simulink model "jumeau_banc_rw"  (R2025b)
settings: Solver=ode23t  StartTime=0.0  StopTime=20  MaxStep=1e-3  RelTol=1e-4
PostLoadFcn:
  | d = fileparts(get_param('jumeau_banc_rw', 'FileName')); addpath(fullfile(d, 'geometrie'), fullfile(d, 'liaison'), fullfile(d, 'pilotage')); clear d
StartFcn:
  | % Jumeau Webots : au lancement, MATLAB envoie les paramètres du Model Workspace à Webots, qui remet le banc en
  | % position de départ, puis ouvre la liaison de télémétrie et la liaison de commande (liaison/pont_banc.m).
  | if strcmp(get_param('jumeau_banc_rw/Procédé', 'LabelModeActiveChoice'), 'Webots')
  |     pont_banc('ouvrir', getVariable(get_param('jumeau_banc_rw', 'ModelWorkspace'), 'config_jumeau'));
  | end
  | pilotage_banc('depart');   % interface de pilotage : nouveau lancement
StopFcn:
  | pont_banc('fermer');
  | pilotage_banc('fin');
model workspace (MATLAB code in the model file):
  | %% Jumeau numérique du banc de stabilisation à 4 roues de réaction (version 3) : paramètres
  | % Ce code est enregistré dans le modèle (Model Explorer > jumeau_banc_rw > Model Workspace).
  | % Origine : (CAO) CAO du banc version 3, (M) mesuré sur le matériel, (F) fiche technique, (Fw) firmware,
  | % (H) hypothèse à mesurer sur le banc. Masses et inerties des pièces : dans chaque bloc de pièce.
  | 
  | %% Montage de l'essai
  | pivot_mm = 25;              % position du pivot de tangage sur le corps : 25, 24, 16, 8, 0, -8 mm (25 : banc équilibré, rangée +24 et paliers remontés de 1 mm)
  | blocage_roulis = 0;         % goupille de blocage : 1 = axe bloqué à 0°, 0 = axe libre
  | blocage_tangage = 0;
  | angle0_roulis_deg = 2;      % position de départ (mise à 0 si l'axe est bloqué)
  | angle0_tangage_deg = -1;
  | g = 9.81;                   % m/s²
  | 
  | %% Pupitre : pilotage manuel des 4 ESC
  | essai_t = 1;                % s, instant de l'échelon d'essai ajouté aux curseurs
  | essai_echelon_us = [0 0 0 0];   % µs, échelon d'essai sur chaque ESC (0 : aucun)
  | 
  | %% Alimentation des ESC
  | V_alim = 12;                % V, alimentation de labo (H : tension réglée)
  | 
  | %% ESC Brushless 30A bidirectionnels (x4)
  | f_trame_esc = 50;           % Hz, une impulsion toutes les 20 ms (Fw : LEDC 50 Hz)
  | imp_neutre = 1500;          % µs, neutre (testé sur le banc)
  | imp_min = 1000;             % µs (Fw)
  | imp_max = 2000;             % µs (Fw)
  | zone_morte_us = 0;          % µs autour du neutre (H)
  | tau_esc = 2e-3;             % s, temps de réponse de l'ESC (H)
  | armement_actif = 1;         % 1 : l'ESC ne pilote le moteur qu'après t_armement au neutre
  | t_armement = 1;             % s (H)
  | fenetre_armement_us = 25;   % µs, écart au neutre accepté pendant l'armement (H)
  | sens_moteurs = [1 1 1 1];   % +1 : au-dessus du neutre, la roue tourne dans le sens +axe (vers l'extérieur) (H : ordre des phases)
  | 
  | %% Moteurs A2212 1400 KV (x4), modèle équivalent continu
  | KV = 1400;                  % tr/min/V (F)
  | Ke = 60/(2*pi*KV);          % V.s/rad
  | Kt = Ke;                    % N.m/A
  | R_moteur = 0.08;            % ohm (H)
  | L_moteur = 30e-6;           % H (H)
  | f_roue = 5e-6;              % N.m.s/rad, frottement visqueux des roulements du moteur (H)
  | 
  | %% Cardan
  | butee_deg = 20;             % débattement de chaque axe (CAO)
  | k_butee = 20;               % N.m/rad, contact goupille-lumière (H)
  | c_butee = 0.2;              % N.m.s/rad (H)
  | b_cardan = 1e-4;            % N.m.s/rad, frottement des roulements 625 (H)
  | k_cables = 0;               % N.m/rad, raideur des deux câbles vers la table (H)
  | 
  | %% BNO055 (mode fusion)
  | T_bno = 0.01;               % s, données de fusion à 100 Hz (F)
  | bruit_bno = 1;              % 1 : bruit de mesure, 0 : capteur parfait
  | sigma_angle_deg = 0.05;     % ° (H)
  | sigma_gyro_dps = 0.1;       % °/s (H)
  | sigma_acc = 0.02;           % m/s² (H)
  | R_montage_bno = eye(3);     % axes du capteur dans le repère du dispositif : eye(3) = remappage AXIS_MAP réglé
  |                             % (la carte est tournée de 90° dans la CAO)
  | 
  | %% Capteurs de vitesse TCRT5000 (x4) : un front à chaque rayon du disque
  | n_rayons = 4;               % rayons du disque vus par tour (CAO : disque d'origine)
  | T_tcrt = 1e-3;              % s, pas de calcul du capteur (les fronts sont datés par interpolation, comme un chronomètre en µs)
  | t_arret_tcrt = 0.2;         % s sans front : la vitesse mesurée retombe à 0 (Fw, à fixer)
  | 
  | %% Pont vers le jumeau Webots (et, plus tard, vers l'ESP32 du banc réel)
  | T_pont = 0.01;              % s, une trame de commande et une trame de télémétrie toutes les 10 ms
  | 
  | %% Essai : maintien au départ et perturbation
  | t_lacher = 2;                % s, le dispositif est tenu à la main à sa position de départ jusqu'à cet instant (0 : libre dès le départ)
  | k_main = 5;                  % N.m/rad, raideur de la main qui tient le dispositif
  | c_main = 0.3;                % N.m.s/rad, son amortissement
  | perturbation_t = 7;          % s, instant de la poussée d'essai
  | perturbation_duree = 0.2;    % s
  | perturbation_couple = [0.02 0.02];   % N.m, couple de la poussée sur [roulis tangage], programmée (0 : aucune ; l'interface de pilotage en ajoute)
  | 
  | %% Grandeurs dérivées
  | assert(any(pivot_mm == [25 24 16 8 0 -8]), 'pivot_mm : 25, 24, 16, 8, 0, -8');
  | q0_deg = [angle0_roulis_deg angle0_tangage_deg] .* ([blocage_roulis blocage_tangage] == 0);
  | config_jumeau = [pivot_mm; blocage_roulis; blocage_tangage; q0_deg(:); V_alim; f_trame_esc; imp_neutre; imp_min; imp_max; ...
  |     zone_morte_us; tau_esc; armement_actif; t_armement; fenetre_armement_us; sens_moteurs(:); Ke; Kt; R_moteur; L_moteur; ...
  |     f_roue; butee_deg; k_butee; c_butee; b_cardan; k_cables; g; T_bno; bruit_bno; sigma_angle_deg; sigma_gyro_dps; ...
  |     sigma_acc; n_rayons; t_arret_tcrt; T_tcrt; R_montage_bno(:); T_pont; t_lacher; k_main; c_main];   % 51 valeurs envoyées au jumeau Webots au lancement
  | 
  | %% Commande bas niveau : une boucle de vitesse par roue, avec observateur CFO (méthode du TP2, ramenée à la vitesse)
  | J_roue = 1.562e-4;          % kg.m², inertie d'une roue autour de son axe : disque, vis, cloche du moteur (CAO)
  | T_cbn = 1/f_trame_esc;      % s, période de calcul de la commande : celle des ESC, qui ne lisent qu'une impulsion toutes les 20 ms
  | wc_roue = [10 10 10 10];    % rad/s, rapidité du suivi de vitesse de chaque roue (pôle de l'erreur en -wc)
  | wo_roue = [5 5 5 5];        % rad/s, rapidité du CFO de chaque roue (pôles en -wo et -4 wo) ; au-delà de 10, il devient instable à 20 ms
  | imp_cmd_min = 1375;         % µs, limites des impulsions commandées : vitesse conseillée des disques, 3 900 tr/min
  | imp_cmd_max = 1625;         % µs
  | w_aveugle = 45;             % rad/s, en dessous (vitesse du modèle), le TCRT5000 voit mal la roue : le CFO ne se corrige plus sur la mesure
  | 
  | %% Consigne d'essai des roues : ajoutée à la consigne qui vient de la conversion (0 tant qu'elle est vide)
  | essai_roue_t1 = 2;                  % s, départ vers le premier palier
  | essai_roue_vitesse1 = [0 0 0 0];  % rad/s, premier palier de chaque roue (0 : la roue reste à l'arrêt)
  | essai_roue_t2 = 6;                  % s, départ vers le second palier
  | essai_roue_vitesse2 = [0 0 0 0];    % rad/s, second palier de chaque roue
  | essai_roue_acc = 300;               % rad/s², pente des rampes entre les paliers
  | 
  | %% Commande bas niveau : grandeurs calculées
  | % modèle local d'une roue : d(omega)/dt = -a1 omega + a0 V + d
  | a0_roue = Kt/(R_moteur*J_roue) * [1 1 1 1];                % rad/s² par volt
  | a1_roue = (Kt*Ke/R_moteur + f_roue)/J_roue * [1 1 1 1];    % 1/s
  | K_roue = wc_roue - a1_roue;                                % retour d'état : erreur en -(a1 + K) = -wc
  | l1_roue = 5*wo_roue;                                       % CFO
  | lambda_roue = 4/5*wo_roue;
  | 
  | %% Référence : angles demandés au dispositif, en polynômes de degré 5 entre deux paliers
  | ref_t = [2 12];              % s, instant de départ vers chaque palier
  | ref_roulis_deg = [0 5];      % °, roulis demandé à chaque palier
  | ref_tangage_deg = [0 0];     % °, tangage demandé à chaque palier
  | ref_duree = 1.5;             % s, durée du passage d'un palier au suivant
  | 
  | %% Commande haut niveau : une boucle par axe [roulis tangage], placement de pôles basé sur l'observateur CFO (TP2)
  | T_chn = T_cbn;               % s, période de calcul : celle de la commande bas niveau et des ESC
  | t_depart = t_lacher;         % s, mise en marche de la commande : au moment où la main lâche le dispositif
  | wc_axe = [4 4];              % rad/s, rapidité du suivi d'angle de chaque axe
  | xi_axe = [1 1];              % amortissement
  | wo_axe = [3 3];              % rad/s, rapidité du CFO de chaque axe (pôles en -wo et -4 wo, double) ; au-delà de 4, le couple s'agite
  | desat_active = 0;            % 1 : la référence est décalée pour ramener les roues vers leur vitesse de repos
  | T_desat = 5;                 % s, constante de temps de ce retour
  | desat_max_deg = 15;          % °, décalage maximal de la référence
  | 
  | %% Conversion : couples des deux axes vers les 4 roues
  | w_repos = 200;               % rad/s, vitesse de repos des 4 roues : elles tournent toujours, le TCRT5000 les voit toujours
  | t_roues = t_armement + 0.2;  % s, mise en rotation des roues, une fois les ESC armés
  | acc_roue_max = 300;          % rad/s², accélération maximale demandée à une roue
  | w_roue_min = 60;             % rad/s, vitesses limites demandées à une roue
  | w_roue_max = 400;            % rad/s (disques : 3 900 tr/min conseillés, soit 408 rad/s)
  | 
  | %% Masses et inerties utilisées par la commande (CAO du banc version 3)
  | m_disp = 1.2615;             % kg, dispositif et ses 4 roues
  | zG_disp = 24.977e-3;         % m, hauteur de son centre de masse sur le corps (le pivot est à pivot_mm)
  | Ixx_disp_24 = 8.2684e-3;     % kg.m², inertie du dispositif autour du roulis, pivot à +24 mm
  | Iyy_disp_24 = 8.2786e-3;     % kg.m², autour du tangage, pivot à +24 mm
  | m_croix = 0.0755;            % kg, croisillon et paliers (ne tournent qu'en roulis)
  | zG_croix = 0.257e-3;         % m, hauteur de leur centre de masse au-dessus de l'axe de roulis
  | Ixx_croix = 2.073e-4;        % kg.m²
  | 
  | %% Commande haut niveau et conversion : grandeurs calculées
  | % modèle local d'un axe : d²(theta)/dt² = -a1 d(theta)/dt + a0 C + d, avec C le couple demandé aux roues
  | hz = zG_disp - pivot_mm/1000;                                    % m, centre de masse du dispositif au-dessus du pivot
  | I_axe = [Ixx_disp_24 + Ixx_croix, Iyy_disp_24] + m_disp*(hz^2 - (zG_disp - 0.024)^2) - 2*J_roue;   % kg.m²
  | mgh_axe = g*[m_disp*hz + m_croix*zG_croix, m_disp*hz];           % N.m/rad, couple de pesanteur par radian d'inclinaison
  | a0_axe = 1./I_axe;                                               % rad/s² par N.m
  | a1_axe = b_cardan./I_axe;                                        % 1/s
  | k1_axe = wc_axe.^2;                                              % retour d'état : s² + 2 xi wc s + wc²
  | k2_axe = 2*xi_axe.*wc_axe - a1_axe;
  | l1_axe = 9*wo_axe;                                               % CFO du TP2
  | l2_axe = 12*wo_axe.^2;
  | lambda_axe = 4/3*wo_axe;
  | C_max = 2*J_roue*cosd(45)*acc_roue_max;                          % N.m, couple maximal demandé sur un axe
  | k_desat = desat_active.*sign(mgh_axe + (mgh_axe == 0))./(max(abs(mgh_axe), 1e-3)*T_desat);            % rad par N.m.s
  | sx_roues = [1 -1 -1 1];                                          % signe de cos(45°, 135°, 225°, 315°) : part de chaque roue sur le roulis
  | sy_roues = [1 1 -1 -1];                                          % signe de sin : part sur le tangage
  | M_conv = -[sx_roues(:) sy_roues(:)]/(4*J_roue*cosd(45));         % accélération des 4 roues pour un couple [roulis; tangage]
  | 
  | %% Perception : des mesures à l'état du banc
  | T_perception = T_bno;        % s, période de calcul : celle du BNO055
  | tau_desequilibre = 2;        % s, constante de temps du filtre du couple extérieur et du déséquilibre
  | 
  | %% Pilotage par l'interface (pilotage/pilote_banc.m)
  | manche_max_deg = 15;         % °, limite de sécurité de l'inclinaison demandée par le manche (l'interface règle l'amplitude)
  | w_manche = 3;                % rad/s, rapidité avec laquelle la référence rejoint le manche (second ordre critique)
  | T_affichage = 0.1;           % s, rafraîchissement de l'interface
undefined symbols (not defined in the file): DiscIntNeverNeededParam, X, Y, Z
libraries: sm_lib x256, nesl_utility x24, simulink x7
(part 8 of 8)

== system jumeau_banc_rw/Procédé/Jumeau Simscape/Mécanique (CAO version 3)/Module de roue 4 (315°)/Rotor 4 (disque, vis, rotor A2212) ==
  A2212 rotor (roue 4) : sm_lib/Body Elements/File Solid  Description=|  ExtGeomFileName=A2212_rotor.stl  UnitType=Custom  ExtGeomFileUnits=mm  StepReaderType=HEX  ExportConvexHullGeometry=off  InertiaType=Custom  BasedOnType=DensityFromFile  Density=1000  DensityUnits=kg/m^3  Mass=0.016827871  MassUnits=kg  CenterOfMass=[2.4267094e-06 -3.2856014e-08 0.015974753]  CenterOfMassUnits=m  MomentsOfInertia=[1.7900011e-06 1.7901749e-06 1.9632852e-06]  MomentsOfInertiaUnits=kg*m^2  ProductsOfInertia=[3.6666561e-12 -1.1397813e-09 -5.9134076e-14]  ProductsOfInertiaUnits=kg*m^2  GraphicType=FromGeometry  MarkerShape=Sphere  MarkerSize=10  GraphicVisPropType=SimpleVisualProperties  GraphicDiffuseColor=[0.549 0.549 0.549]  GraphicOpacity=1  GraphicSpecularColor=[0.5 0.5 0.5 1.0]  GraphicAmbientColor=[0.15 0.15 0.15 1.0]  GraphicEmissiveColor=[0.0 0.0 0.0 1.0]  GraphicShininess=75  DoExposeReferenceFrame=on  SerializedFrames=<Frames/>
      | Pièce CAO : A2212 rotor (roue 4) (A2212_rotor)
      | Masse 16.83 g : cloche aluminium, 14 aimants NdFeB 7500 kg/m³, arbre, vis pointeau et circlip acier.
      | Centre de masse et inertie : calculés sur la géométrie de la CAO.
  Pose A2212 rotor (roue 4) : sm_lib/Frames and Transforms/Rigid Transform  RotationMethod=RotationMatrix  FollAlignAxisA=+X  BaseAlignAxisA=+Y  FollAlignAxisB=+Y  BaseAlignAxisB=+Z  RotationStandardAxis=+Z  RotationAngle=0  RotationAngleUnits=deg  RotationArbitraryAxis=[0 0 1]  RotationSequenceAxes=FollowerAxes  RotationSequence=XYX  RotationSequenceAngles=[0 0 0]  RotationSequenceAnglesUnits=deg  RotationMatrix=[0 -1 0;1 0 0;0 0 1]  Quaternion=[1 0 0 0]  TranslationMethod=Cartesian  TranslationCartesianOffset=[0 0.001192 86]  TranslationCartesianOffsetUnits=mm  TranslationStandardAxis=+Z  TranslationStandardOffset=0  TranslationStandardOffsetUnits=m  TranslationROffset=0  TranslationROffsetUnits=m  TranslationThetaOffset=0  TranslationThetaOffsetUnits=deg  TranslationZOffset=0  TranslationZOffsetUnits=m
  Pose disque-1 (roue 4) : sm_lib/Frames and Transforms/Rigid Transform  RotationMethod=RotationMatrix  FollAlignAxisA=+X  BaseAlignAxisA=+Y  FollAlignAxisB=+Y  BaseAlignAxisB=+Z  RotationStandardAxis=+Z  RotationAngle=0  RotationAngleUnits=deg  RotationArbitraryAxis=[0 0 1]  RotationSequenceAxes=FollowerAxes  RotationSequence=XYX  RotationSequenceAngles=[0 0 0]  RotationSequenceAnglesUnits=deg  RotationMatrix=[0 -1 0;1 0 0;0 0 1]  Quaternion=[1 0 0 0]  TranslationMethod=Cartesian  TranslationCartesianOffset=[0 0 116.7]  TranslationCartesianOffsetUnits=mm  TranslationStandardAxis=+Z  TranslationStandardOffset=0  TranslationStandardOffsetUnits=m  TranslationROffset=0  TranslationROffsetUnits=m  TranslationThetaOffset=0  TranslationThetaOffsetUnits=deg  TranslationZOffset=0  TranslationZOffsetUnits=m
  Pose ecrous-1 (roue 4) : sm_lib/Frames and Transforms/Rigid Transform  RotationMethod=RotationMatrix  FollAlignAxisA=+X  BaseAlignAxisA=+Y  FollAlignAxisB=+Y  BaseAlignAxisB=+Z  RotationStandardAxis=+Z  RotationAngle=0  RotationAngleUnits=deg  RotationArbitraryAxis=[0 0 1]  RotationSequenceAxes=FollowerAxes  RotationSequence=XYX  RotationSequenceAngles=[0 0 0]  RotationSequenceAnglesUnits=deg  RotationMatrix=[0 -1 0;1 0 0;0 0 1]  Quaternion=[1 0 0 0]  TranslationMethod=Cartesian  TranslationCartesianOffset=[0 -55 110.7]  TranslationCartesianOffsetUnits=mm  TranslationStandardAxis=+Z  TranslationStandardOffset=0  TranslationStandardOffsetUnits=m  TranslationROffset=0  TranslationROffsetUnits=m  TranslationThetaOffset=0  TranslationThetaOffsetUnits=deg  TranslationZOffset=0  TranslationZOffsetUnits=m
  Pose ecrous-2 (roue 4) : sm_lib/Frames and Transforms/Rigid Transform  RotationMethod=RotationMatrix  FollAlignAxisA=+X  BaseAlignAxisA=+Y  FollAlignAxisB=+Y  BaseAlignAxisB=+Z  RotationStandardAxis=+Z  RotationAngle=0  RotationAngleUnits=deg  RotationArbitraryAxis=[0 0 1]  RotationSequenceAxes=FollowerAxes  RotationSequence=XYX  RotationSequenceAngles=[0 0 0]  RotationSequenceAnglesUnits=deg  RotationMatrix=[0 -1 0;1 0 0;0 0 1]  Quaternion=[1 0 0 0]  TranslationMethod=Cartesian  TranslationCartesianOffset=[55 0 110.7]  TranslationCartesianOffsetUnits=mm  TranslationStandardAxis=+Z  TranslationStandardOffset=0  TranslationStandardOffsetUnits=m  TranslationROffset=0  TranslationROffsetUnits=m  TranslationThetaOffset=0  TranslationThetaOffsetUnits=deg  TranslationZOffset=0  TranslationZOffsetUnits=m
  Pose ecrous-3 (roue 4) : sm_lib/Frames and Transforms/Rigid Transform  RotationMethod=RotationMatrix  FollAlignAxisA=+X  BaseAlignAxisA=+Y  FollAlignAxisB=+Y  BaseAlignAxisB=+Z  RotationStandardAxis=+Z  RotationAngle=0  RotationAngleUnits=deg  RotationArbitraryAxis=[0 0 1]  RotationSequenceAxes=FollowerAxes  RotationSequence=XYX  RotationSequenceAngles=[0 0 0]  RotationSequenceAnglesUnits=deg  RotationMatrix=[0 -1 0;1 0 0;0 0 1]  Quaternion=[1 0 0 0]  TranslationMethod=Cartesian  TranslationCartesianOffset=[-55 0 110.7]  TranslationCartesianOffsetUnits=mm  TranslationStandardAxis=+Z  TranslationStandardOffset=0  TranslationStandardOffsetUnits=m  TranslationROffset=0  TranslationROffsetUnits=m  TranslationThetaOffset=0  TranslationThetaOffsetUnits=deg  TranslationZOffset=0  TranslationZOffsetUnits=m
  Pose ecrous-4 (roue 4) : sm_lib/Frames and Transforms/Rigid Transform  RotationMethod=RotationMatrix  FollAlignAxisA=+X  BaseAlignAxisA=+Y  FollAlignAxisB=+Y  BaseAlignAxisB=+Z  RotationStandardAxis=+Z  RotationAngle=0  RotationAngleUnits=deg  RotationArbitraryAxis=[0 0 1]  RotationSequenceAxes=FollowerAxes  RotationSequence=XYX  RotationSequenceAngles=[0 0 0]  RotationSequenceAnglesUnits=deg  RotationMatrix=[0 -1 0;1 0 0;0 0 1]  Quaternion=[1 0 0 0]  TranslationMethod=Cartesian  TranslationCartesianOffset=[0 55 110.7]  TranslationCartesianOffsetUnits=mm  TranslationStandardAxis=+Z  TranslationStandardOffset=0  TranslationStandardOffsetUnits=m  TranslationROffset=0  TranslationROffsetUnits=m  TranslationThetaOffset=0  TranslationThetaOffsetUnits=deg  TranslationZOffset=0  TranslationZOffsetUnits=m
  Pose vis10-1 (roue 4) : sm_lib/Frames and Transforms/Rigid Transform  RotationMethod=RotationMatrix  FollAlignAxisA=+X  BaseAlignAxisA=+Y  FollAlignAxisB=+Y  BaseAlignAxisB=+Z  RotationStandardAxis=+Z  RotationAngle=0  RotationAngleUnits=deg  RotationArbitraryAxis=[0 0 1]  RotationSequenceAxes=FollowerAxes  RotationSequence=XYX  RotationSequenceAngles=[0 0 0]  RotationSequenceAnglesUnits=deg  RotationMatrix=[0 -1 0;1 0 0;0 0 1]  Quaternion=[1 0 0 0]  TranslationMethod=Cartesian  TranslationCartesianOffset=[55 0 111.2]  TranslationCartesianOffsetUnits=mm  TranslationStandardAxis=+Z  TranslationStandardOffset=0  TranslationStandardOffsetUnits=m  TranslationROffset=0  TranslationROffsetUnits=m  TranslationThetaOffset=0  TranslationThetaOffsetUnits=deg  TranslationZOffset=0  TranslationZOffsetUnits=m
  Pose vis10-2 (roue 4) : sm_lib/Frames and Transforms/Rigid Transform  RotationMethod=RotationMatrix  FollAlignAxisA=+X  BaseAlignAxisA=+Y  FollAlignAxisB=+Y  BaseAlignAxisB=+Z  RotationStandardAxis=+Z  RotationAngle=0  RotationAngleUnits=deg  RotationArbitraryAxis=[0 0 1]  RotationSequenceAxes=FollowerAxes  RotationSequence=XYX  RotationSequenceAngles=[0 0 0]  RotationSequenceAnglesUnits=deg  RotationMatrix=[0 -1 0;1 0 0;0 0 1]  Quaternion=[1 0 0 0]  TranslationMethod=Cartesian  TranslationCartesianOffset=[-55 0 111.2]  TranslationCartesianOffsetUnits=mm  TranslationStandardAxis=+Z  TranslationStandardOffset=0  TranslationStandardOffsetUnits=m  TranslationROffset=0  TranslationROffsetUnits=m  TranslationThetaOffset=0  TranslationThetaOffsetUnits=deg  TranslationZOffset=0  TranslationZOffsetUnits=m
  Pose vis20-1 (roue 4) : sm_lib/Frames and Transforms/Rigid Transform  RotationMethod=RotationMatrix  FollAlignAxisA=+X  BaseAlignAxisA=+Y  FollAlignAxisB=+Y  BaseAlignAxisB=+Z  RotationStandardAxis=+Z  RotationAngle=0  RotationAngleUnits=deg  RotationArbitraryAxis=[0 0 1]  RotationSequenceAxes=FollowerAxes  RotationSequence=XYX  RotationSequenceAngles=[0 0 0]  RotationSequenceAnglesUnits=deg  RotationMatrix=[0 -1 0;1 0 0;0 0 1]  Quaternion=[1 0 0 0]  TranslationMethod=Cartesian  TranslationCartesianOffset=[0 55 101.2]  TranslationCartesianOffsetUnits=mm  TranslationStandardAxis=+Z  TranslationStandardOffset=0  TranslationStandardOffsetUnits=m  TranslationROffset=0  TranslationROffsetUnits=m  TranslationThetaOffset=0  TranslationThetaOffsetUnits=deg  TranslationZOffset=0  TranslationZOffsetUnits=m
  Pose vis20-2 (roue 4) : sm_lib/Frames and Transforms/Rigid Transform  RotationMethod=RotationMatrix  FollAlignAxisA=+X  BaseAlignAxisA=+Y  FollAlignAxisB=+Y  BaseAlignAxisB=+Z  RotationStandardAxis=+Z  RotationAngle=0  RotationAngleUnits=deg  RotationArbitraryAxis=[0 0 1]  RotationSequenceAxes=FollowerAxes  RotationSequence=XYX  RotationSequenceAngles=[0 0 0]  RotationSequenceAnglesUnits=deg  RotationMatrix=[0 -1 0;1 0 0;0 0 1]  Quaternion=[1 0 0 0]  TranslationMethod=Cartesian  TranslationCartesianOffset=[0 -55 99.853166]  TranslationCartesianOffsetUnits=mm  TranslationStandardAxis=+Z  TranslationStandardOffset=0  TranslationStandardOffsetUnits=m  TranslationROffset=0  TranslationROffsetUnits=m  TranslationThetaOffset=0  TranslationThetaOffsetUnits=deg  TranslationZOffset=0  TranslationZOffsetUnits=m
  disque-1 (roue 4) : sm_lib/Body Elements/File Solid  Description=|  ExtGeomFileName=disque.stl  UnitType=Custom  ExtGeomFileUnits=mm  StepReaderType=HEX  ExportConvexHullGeometry=off  InertiaType=Custom  BasedOnType=DensityFromFile  Density=1000  DensityUnits=kg/m^3  Mass=0.027339457  MassUnits=kg  CenterOfMass=[3.5840173e-18 -4.1025221e-18 0.00225]  CenterOfMassUnits=m  MomentsOfInertia=[3.0147281e-05 3.0147281e-05 6.0202291e-05]  MomentsOfInertiaUnits=kg*m^2  ProductsOfInertia=[3.9369464e-23 -4.3624716e-23 -7.0860886e-22]  ProductsOfInertiaUnits=kg*m^2  GraphicType=FromGeometry  MarkerShape=Sphere  MarkerSize=10  GraphicVisPropType=SimpleVisualProperties  GraphicDiffuseColor=[0.769 0.306 0.322]  GraphicOpacity=1  GraphicSpecularColor=[0.5 0.5 0.5 1.0]  GraphicAmbientColor=[0.15 0.15 0.15 1.0]  GraphicEmissiveColor=[0.0 0.0 0.0 1.0]  GraphicShininess=75  DoExposeReferenceFrame=on  SerializedFrames=<Frames/>
      | Pièce CAO : disque-1 (roue 4) (disque)
      | Masse 27.34 g : PLA, plein × 0,9 (même hypothèse que le TP1), 1116 kg/m³.
      | Centre de masse et inertie : calculés sur la géométrie de la CAO.
  ecrous-1 (roue 4) : sm_lib/Body Elements/File Solid  Description=|  ExtGeomFileName=ecrous.stl  UnitType=Custom  ExtGeomFileUnits=mm  StepReaderType=HEX  ExportConvexHullGeometry=off  InertiaType=Custom  BasedOnType=DensityFromFile  Density=1000  DensityUnits=kg/m^3  Mass=0.0027655409  MassUnits=kg  CenterOfMass=[3.1829158e-19 0 0.003]  CenterOfMassUnits=m  MomentsOfInertia=[3.7203439e-08 3.7203439e-08 5.7813632e-08]  MomentsOfInertiaUnits=kg*m^2  ProductsOfInertia=[-1.9726372e-40 -8.2344948e-41 -7.5517615e-41]  ProductsOfInertiaUnits=kg*m^2  GraphicType=FromGeometry  MarkerShape=Sphere  MarkerSize=10  GraphicVisPropType=SimpleVisualProperties  GraphicDiffuseColor=[0.439 0.439 0.439]  GraphicOpacity=1  GraphicSpecularColor=[0.5 0.5 0.5 1.0]  GraphicAmbientColor=[0.15 0.15 0.15 1.0]  GraphicEmissiveColor=[0.0 0.0 0.0 1.0]  GraphicShininess=75  DoExposeReferenceFrame=on  SerializedFrames=<Frames/>
      | Pièce CAO : ecrous-1 (roue 4) (ecrous)
      | Masse 2.77 g : acier, 7850 kg/m³.
      | Centre de masse et inertie : calculés sur la géométrie de la CAO.
  ecrous-2 (roue 4) : sm_lib/Body Elements/File Solid  Description=|  ExtGeomFileName=ecrous.stl  UnitType=Custom  ExtGeomFileUnits=mm  StepReaderType=HEX  ExportConvexHullGeometry=off  InertiaType=Custom  BasedOnType=DensityFromFile  Density=1000  DensityUnits=kg/m^3  Mass=0.0027655409  MassUnits=kg  CenterOfMass=[3.1829158e-19 0 0.003]  CenterOfMassUnits=m  MomentsOfInertia=[3.7203439e-08 3.7203439e-08 5.7813632e-08]  MomentsOfInertiaUnits=kg*m^2  ProductsOfInertia=[-1.9726372e-40 -8.2344948e-41 -7.5517615e-41]  ProductsOfInertiaUnits=kg*m^2  GraphicType=FromGeometry  MarkerShape=Sphere  MarkerSize=10  GraphicVisPropType=SimpleVisualProperties  GraphicDiffuseColor=[0.439 0.439 0.439]  GraphicOpacity=1  GraphicSpecularColor=[0.5 0.5 0.5 1.0]  GraphicAmbientColor=[0.15 0.15 0.15 1.0]  GraphicEmissiveColor=[0.0 0.0 0.0 1.0]  GraphicShininess=75  DoExposeReferenceFrame=on  SerializedFrames=<Frames/>
      | Pièce CAO : ecrous-2 (roue 4) (ecrous)
      | Masse 2.77 g : acier, 7850 kg/m³.
      | Centre de masse et inertie : calculés sur la géométrie de la CAO.
  ecrous-3 (roue 4) : sm_lib/Body Elements/File Solid  Description=|  ExtGeomFileName=ecrous.stl  UnitType=Custom  ExtGeomFileUnits=mm  StepReaderType=HEX  ExportConvexHullGeometry=off  InertiaType=Custom  BasedOnType=DensityFromFile  Density=1000  DensityUnits=kg/m^3  Mass=0.0027655409  MassUnits=kg  CenterOfMass=[3.1829158e-19 0 0.003]  CenterOfMassUnits=m  MomentsOfInertia=[3.7203439e-08 3.7203439e-08 5.7813632e-08]  MomentsOfInertiaUnits=kg*m^2  ProductsOfInertia=[-1.9726372e-40 -8.2344948e-41 -7.5517615e-41]  ProductsOfInertiaUnits=kg*m^2  GraphicType=FromGeometry  MarkerShape=Sphere  MarkerSize=10  GraphicVisPropType=SimpleVisualProperties  GraphicDiffuseColor=[0.439 0.439 0.439]  GraphicOpacity=1  GraphicSpecularColor=[0.5 0.5 0.5 1.0]  GraphicAmbientColor=[0.15 0.15 0.15 1.0]  GraphicEmissiveColor=[0.0 0.0 0.0 1.0]  GraphicShininess=75  DoExposeReferenceFrame=on  SerializedFrames=<Frames/>
      | Pièce CAO : ecrous-3 (roue 4) (ecrous)
      | Masse 2.77 g : acier, 7850 kg/m³.
      | Centre de masse et inertie : calculés sur la géométrie de la CAO.
  ecrous-4 (roue 4) : sm_lib/Body Elements/File Solid  Description=|  ExtGeomFileName=ecrous.stl  UnitType=Custom  ExtGeomFileUnits=mm  StepReaderType=HEX  ExportConvexHullGeometry=off  InertiaType=Custom  BasedOnType=DensityFromFile  Density=1000  DensityUnits=kg/m^3  Mass=0.0027655409  MassUnits=kg  CenterOfMass=[3.1829158e-19 0 0.003]  CenterOfMassUnits=m  MomentsOfInertia=[3.7203439e-08 3.7203439e-08 5.7813632e-08]  MomentsOfInertiaUnits=kg*m^2  ProductsOfInertia=[-1.9726372e-40 -8.2344948e-41 -7.5517615e-41]  ProductsOfInertiaUnits=kg*m^2  GraphicType=FromGeometry  MarkerShape=Sphere  MarkerSize=10  GraphicVisPropType=SimpleVisualProperties  GraphicDiffuseColor=[0.439 0.439 0.439]  GraphicOpacity=1  GraphicSpecularColor=[0.5 0.5 0.5 1.0]  GraphicAmbientColor=[0.15 0.15 0.15 1.0]  GraphicEmissiveColor=[0.0 0.0 0.0 1.0]  GraphicShininess=75  DoExposeReferenceFrame=on  SerializedFrames=<Frames/>
      | Pièce CAO : ecrous-4 (roue 4) (ecrous)
      | Masse 2.77 g : acier, 7850 kg/m³.
      | Centre de masse et inertie : calculés sur la géométrie de la CAO.
  vis10-1 (roue 4) : sm_lib/Body Elements/File Solid  Description=|  ExtGeomFileName=vis10.stl  UnitType=Custom  ExtGeomFileUnits=mm  StepReaderType=HEX  ExportConvexHullGeometry=off  InertiaType=Custom  BasedOnType=DensityFromFile  Density=1000  DensityUnits=kg/m^3  Mass=0.003481639  MassUnits=kg  CenterOfMass=[4.3728344e-18 1.1656449e-19 0.0073902526]  CenterOfMassUnits=m  MomentsOfInertia=[6.4384479e-08 6.4384479e-08 1.9106608e-08]  MomentsOfInertiaUnits=kg*m^2  ProductsOfInertia=[-6.8499851e-25 -3.7892566e-23 -1.212724e-24]  ProductsOfInertiaUnits=kg*m^2  GraphicType=FromGeometry  MarkerShape=Sphere  MarkerSize=10  GraphicVisPropType=SimpleVisualProperties  GraphicDiffuseColor=[0.439 0.439 0.439]  GraphicOpacity=1  GraphicSpecularColor=[0.5 0.5 0.5 1.0]  GraphicAmbientColor=[0.15 0.15 0.15 1.0]  GraphicEmissiveColor=[0.0 0.0 0.0 1.0]  GraphicShininess=75  DoExposeReferenceFrame=on  SerializedFrames=<Frames/>
      | Pièce CAO : vis10-1 (roue 4) (vis10)
      | Masse 3.48 g : acier, 7850 kg/m³.
      | Centre de masse et inertie : calculés sur la géométrie de la CAO.
  vis10-2 (roue 4) : sm_lib/Body Elements/File Solid  Description=|  ExtGeomFileName=vis10.stl  UnitType=Custom  ExtGeomFileUnits=mm  StepReaderType=HEX  ExportConvexHullGeometry=off  InertiaType=Custom  BasedOnType=DensityFromFile  Density=1000  DensityUnits=kg/m^3  Mass=0.003481639  MassUnits=kg  CenterOfMass=[4.3728344e-18 1.1656449e-19 0.0073902526]  CenterOfMassUnits=m  MomentsOfInertia=[6.4384479e-08 6.4384479e-08 1.9106608e-08]  MomentsOfInertiaUnits=kg*m^2  ProductsOfInertia=[-6.8499851e-25 -3.7892566e-23 -1.212724e-24]  ProductsOfInertiaUnits=kg*m^2  GraphicType=FromGeometry  MarkerShape=Sphere  MarkerSize=10  GraphicVisPropType=SimpleVisualProperties  GraphicDiffuseColor=[0.439 0.439 0.439]  GraphicOpacity=1  GraphicSpecularColor=[0.5 0.5 0.5 1.0]  GraphicAmbientColor=[0.15 0.15 0.15 1.0]  GraphicEmissiveColor=[0.0 0.0 0.0 1.0]  GraphicShininess=75  DoExposeReferenceFrame=on  SerializedFrames=<Frames/>
      | Pièce CAO : vis10-2 (roue 4) (vis10)
      | Masse 3.48 g : acier, 7850 kg/m³.
      | Centre de masse et inertie : calculés sur la géométrie de la CAO.
  vis20-1 (roue 4) : sm_lib/Body Elements/File Solid  Description=|  ExtGeomFileName=vis20.stl  UnitType=Custom  ExtGeomFileUnits=mm  StepReaderType=HEX  ExportConvexHullGeometry=off  InertiaType=Custom  BasedOnType=DensityFromFile  Density=1000  DensityUnits=kg/m^3  Mass=0.0064718461  MassUnits=kg  CenterOfMass=[2.390239e-18 -6.2707839e-20 0.012260949]  CenterOfMassUnits=m  MomentsOfInertia=[3.2989031e-07 3.2989031e-07 3.6632652e-08]  MomentsOfInertiaUnits=kg*m^2  ProductsOfInertia=[3.1154167e-24 -1.1458442e-22 -6.862747e-24]  ProductsOfInertiaUnits=kg*m^2  GraphicType=FromGeometry  MarkerShape=Sphere  MarkerSize=10  GraphicVisPropType=SimpleVisualProperties  GraphicDiffuseColor=[0.439 0.439 0.439]  GraphicOpacity=1  GraphicSpecularColor=[0.5 0.5 0.5 1.0]  GraphicAmbientColor=[0.15 0.15 0.15 1.0]  GraphicEmissiveColor=[0.0 0.0 0.0 1.0]  GraphicShininess=75  DoExposeReferenceFrame=on  SerializedFrames=<Frames/>
      | Pièce CAO : vis20-1 (roue 4) (vis20)
      | Masse 6.47 g : acier, 7850 kg/m³.
      | Centre de masse et inertie : calculés sur la géométrie de la CAO.
  vis20-2 (roue 4) : sm_lib/Body Elements/File Solid  Description=|  ExtGeomFileName=vis20.stl  UnitType=Custom  ExtGeomFileUnits=mm  StepReaderType=HEX  ExportConvexHullGeometry=off  InertiaType=Custom  BasedOnType=DensityFromFile  Density=1000  DensityUnits=kg/m^3  Mass=0.0064718461  MassUnits=kg  CenterOfMass=[2.390239e-18 -6.2707839e-20 0.012260949]  CenterOfMassUnits=m  MomentsOfInertia=[3.2989031e-07 3.2989031e-07 3.6632652e-08]  MomentsOfInertiaUnits=kg*m^2  ProductsOfInertia=[3.1154167e-24 -1.1458442e-22 -6.862747e-24]  ProductsOfInertiaUnits=kg*m^2  GraphicType=FromGeometry  MarkerShape=Sphere  MarkerSize=10  GraphicVisPropType=SimpleVisualProperties  GraphicDiffuseColor=[0.439 0.439 0.439]  GraphicOpacity=1  GraphicSpecularColor=[0.5 0.5 0.5 1.0]  GraphicAmbientColor=[0.15 0.15 0.15 1.0]  GraphicEmissiveColor=[0.0 0.0 0.0 1.0]  GraphicShininess=75  DoExposeReferenceFrame=on  SerializedFrames=<Frames/>
      | Pièce CAO : vis20-2 (roue 4) (vis20)
      | Masse 6.47 g : acier, 7850 kg/m³.
      | Centre de masse et inertie : calculés sur la géométrie de la CAO.
  F : PMIOPort  Side=Left
  connections:
  Pose A2212 rotor (roue 4)/LConn1 -- F/RConn1 -- Pose ecrous-2 (roue 4)/LConn1 -- Pose vis10-1 (roue 4)/LConn1 -- Pose vis10-2 (roue 4)/LConn1 -- Pose ecrous-1 (roue 4)/LConn1 -- Pose vis20-1 (roue 4)/LConn1 -- Pose vis20-2 (roue 4)/LConn1 -- Pose ecrous-3 (roue 4)/LConn1 -- Pose disque-1 (roue 4)/LConn1 -- Pose ecrous-4 (roue 4)/LConn1
  Pose A2212 rotor (roue 4)/RConn1 -- A2212 rotor (roue 4)/RConn1
  Pose ecrous-2 (roue 4)/RConn1 -- ecrous-2 (roue 4)/RConn1
  Pose vis10-1 (roue 4)/RConn1 -- vis10-1 (roue 4)/RConn1
  Pose vis10-2 (roue 4)/RConn1 -- vis10-2 (roue 4)/RConn1
  Pose ecrous-1 (roue 4)/RConn1 -- ecrous-1 (roue 4)/RConn1
  Pose vis20-1 (roue 4)/RConn1 -- vis20-1 (roue 4)/RConn1
  Pose vis20-2 (roue 4)/RConn1 -- vis20-2 (roue 4)/RConn1
  Pose ecrous-3 (roue 4)/RConn1 -- ecrous-3 (roue 4)/RConn1
  Pose disque-1 (roue 4)/RConn1 -- disque-1 (roue 4)/RConn1
  Pose ecrous-4 (roue 4)/RConn1 -- ecrous-4 (roue 4)/RConn1

== matlab function jumeau_banc_rw/Procédé/Jumeau Simscape/Capteur BNO055/+ bruit quat ==
  data: q input; qb output; n input
function qb = bruit(q, n)
% Bruit de mesure de l'orientation : une petite rotation n (rad, axes du capteur), de même écart type que celui des
% angles d'Euler. Le BNO055 tire ses angles d'Euler de son quaternion : les deux portent le même bruit, seul leur pas diffère.
d = [1; n(:) / 2];
qb = [q(1)*d(1) - q(2:4).'*d(2:4); q(1)*d(2:4) + d(1)*q(2:4) + cross(q(2:4), d(2:4))];
qb = qb / norm(qb);
if qb(1) < 0, qb = -qb; end

== matlab function jumeau_banc_rw/Perception/Inclinaison x2/Angles du cardan (quaternion) ==
  data: q input; angles output; R_montage_bno parameter
function angles = angles_cardan(q, R_montage_bno)
% Angles de roulis et de tangage du cardan (rad), tirés du quaternion q = [w; x; y; z] du BNO055 (orientation du capteur
% dans le repère fixe). On en tire la verticale vue par le capteur, puis vue par le dispositif (R_montage_bno). Le cardan
% tourne en roulis (axe X), puis en tangage (axe Y) : la verticale vue par le dispositif vaut
% [-cos(roulis) sin(tangage) ; sin(roulis) ; cos(roulis) cos(tangage)]. Le cap du capteur n'intervient pas.
angles = zeros(2, 1);
nq = norm(q);
if nq < 0.5, return, end                       % pas encore de mesure
q = q(:) / nq;
w = q(1); x = q(2); y = q(3); z = q(4);
v = R_montage_bno * [2*(x*z - w*y); 2*(y*z + w*x); 1 - 2*(x^2 + y^2)];
angles = [atan2(v(2), sqrt(v(1)^2 + v(3)^2)); atan2(-v(1), v(3))];

== matlab function jumeau_banc_rw/Perception/Inclinaison x2/Vitesses du cardan (gyroscope) ==
  data: gyro_dps input; vitesses output; angles input; R_montage_bno parameter
function vitesses = vitesses_cardan(gyro_dps, angles, R_montage_bno)
% Vitesses de roulis et de tangage (rad/s), tirées du gyroscope du BNO055 (axes du capteur, ramenés aux axes du dispositif).
% Pour le cardan, la vitesse de rotation vue par le dispositif vaut
% [cos(tangage) d(roulis)/dt ; d(tangage)/dt ; sin(tangage) d(roulis)/dt].
w = R_montage_bno * gyro_dps(:) * pi/180;
c = cos(angles(2)); s = sin(angles(2));
vitesses = [c*w(1) + s*w(3); w(2)];

== matlab function jumeau_banc_rw/Perception/Réserve des roues/Marge aux limites ==
  data: w input; r output; w_roue_min parameter; w_roue_max parameter; w_repos parameter
function r = marge(w, w_roue_min, w_roue_max, w_repos)
% Réserve des roues, de 0 à 1 : 1 quand les 4 roues sont à leur vitesse de repos, 0 quand l'une d'elles atteint une
% limite de vitesse. C'est la part du moment cinétique que les roues peuvent encore absorber.
m = min(min(w(:) - w_roue_min), min(w_roue_max - w(:)));
r = max(0, min(1, m / max(min(w_repos - w_roue_min, w_roue_max - w_repos), 1)));

== matlab function jumeau_banc_rw/Référence/Manche : filtre du second ordre ==
  data: manche input; angle output; angle_programme input; t input; vitesse output; acceleration output; actif output; T_chn parameter; w_manche parameter; manche_max_deg parameter; t_depart parameter
function [angle, vitesse, acceleration, actif] = filtre(manche, angle_programme, t, T_chn, w_manche, manche_max_deg, t_depart)
% Référence donnée par le manche de l'interface de pilotage. manche = [actif ; roulis demandé ; tangage demandé] (°).
% L'angle demandé, borné à manche_max_deg, est suivi par un second ordre critique de pulsation w_manche :
% d²(angle)/dt² = w_manche² (demandé - angle) - 2 w_manche d(angle)/dt. On en tire la vitesse et l'accélération que la
% loi de commande du TP2 demande. Manche inactif, ou dispositif encore tenu (avant t_depart) : le filtre suit la référence
% programmée, sans à-coup au passage au manche.
persistent x v
if isempty(x), x = angle_programme(:); v = zeros(2, 1); end
actif = double(manche(1) > 0.5 && t >= t_depart);
if actif
    c = max(-manche_max_deg, min(manche_max_deg, manche(2:3)));
    a = w_manche^2 * (c(:) - x) - 2 * w_manche * v;
else
    x = angle_programme(:); v = zeros(2, 1); a = zeros(2, 1);
end
angle = x; vitesse = v; acceleration = a;
x = x + T_chn * v;
v = v + T_chn * a;

== matlab function jumeau_banc_rw/Interface de pilotage/Lecture de l'interface ==
  data: t input; manche output; poussee output
function [manche, poussee] = lecture(t)
% Lit l'interface de pilotage (pilotage/pilotage_banc.m) : manche = [actif ; roulis demandé (°) ; tangage demandé (°)],
% poussee = poussée en cours sur [roulis ; tangage] (N.m). Sans interface ouverte : manche inactif, aucune poussée.
coder.extrinsic('pilotage_banc');
s = zeros(5, 1);
s = pilotage_banc('lire', t);
manche = s(1:3);
poussee = s(4:5);

== matlab function jumeau_banc_rw/Tableau de bord/Envoi à l'interface ==
  settings: updateMethod=DISCRETE  sampleTime=T_affichage
  data: angles_deg input; roues input; reserve input; desequilibre_mm input; reference_deg input; poussee input; t input
function envoi(angles_deg, roues, reserve, desequilibre_mm, reference_deg, poussee, t)
% Envoie l'état du banc à l'interface de pilotage (pilotage/pilotage_banc.m), toutes les T_affichage secondes :
% angles et référence [roulis ; tangage] (°), vitesses des 4 roues avec leur signe (rad/s), réserve des roues (0 à 1),
% centre de masse par rapport au pivot [selon X ; selon Y] (mm), poussée en cours (N.m).
coder.extrinsic('pilotage_banc');
pilotage_banc('afficher', t, [angles_deg(:); reference_deg(:); roues(:); reserve; desequilibre_mm(:); poussee(:)]);

== matlab function jumeau_banc_rw/Procédé/Jumeau Simscape/Capteur BNO055/Fusion BNO055 ==
  data: R input; euler output; omega input; a input; gyro output; quat output; acc output; g parameter; R_montage_bno parameter
function [euler, gyro, quat, acc] = fusion(R, omega, a, g, R_montage_bno)
% Ce que la puce calcule en mode fusion, à partir de l'orientation vraie du capteur.
% euler = [cap; roulis; tangage] en degrés (ordre des registres du BNO055), séquence Z-Y-X.
Rs = R * R_montage_bno;                     % axes du capteur dans le repère fixe
w = Rs.' * omega;                           % gyroscope : vitesse angulaire dans les axes du capteur
f = Rs.' * (a - [0; 0; -g]);                % accéléromètre : accélération moins la pesanteur
cap = atan2(Rs(2, 1), Rs(1, 1));
roulis = atan2(Rs(3, 2), Rs(3, 3));
tangage = -asin(max(-1, min(1, Rs(3, 1))));
euler = [cap; roulis; tangage] * 180/pi;
gyro = w * 180/pi;
acc = f;
% quaternion [w; x; y; z] de Rs
t = Rs(1, 1) + Rs(2, 2) + Rs(3, 3);
if t > 0
    q0 = sqrt(1 + t) / 2;
    quat = [q0; (Rs(3, 2) - Rs(2, 3)) / (4*q0); (Rs(1, 3) - Rs(3, 1)) / (4*q0); (Rs(2, 1) - Rs(1, 2)) / (4*q0)];
else
    [~, k] = max([Rs(1, 1) Rs(2, 2) Rs(3, 3)]);
    switch k
        case 1
            r = sqrt(1 + Rs(1, 1) - Rs(2, 2) - Rs(3, 3)) * 2;
            quat = [(Rs(3, 2) - Rs(2, 3)) / r; r/4; (Rs(1, 2) + Rs(2, 1)) / r; (Rs(1, 3) + Rs(3, 1)) / r];
        case 2
            r = sqrt(1 + Rs(2, 2) - Rs(1, 1) - Rs(3, 3)) * 2;
            quat = [(Rs(1, 3) - Rs(3, 1)) / r; (Rs(1, 2) + Rs(2, 1)) / r; r/4; (Rs(2, 3) + Rs(3, 2)) / r];
        otherwise
            r = sqrt(1 + Rs(3, 3) - Rs(1, 1) - Rs(2, 2)) * 2;
            quat = [(Rs(2, 1) - Rs(1, 2)) / r; (Rs(1, 3) + Rs(3, 1)) / r; (Rs(2, 3) + Rs(3, 2)) / r; r/4];
    end
end
if quat(1) < 0, quat = -quat; end

== matlab function jumeau_banc_rw/Procédé/Jumeau Simscape/ESC x4/Armement ==
  data: imp input; arme output; armement_actif parameter; t_armement parameter; fenetre_armement_us parameter; imp_neutre parameter; f_trame_esc parameter
function arme = armement(imp, armement_actif, t_armement, fenetre_armement_us, imp_neutre, f_trame_esc)
% Un ESC ne pilote son moteur qu'après avoir reçu le neutre pendant t_armement depuis sa mise sous tension.
% Tant qu'il n'est pas armé, il bipe et laisse le moteur libre.
persistent duree etat
if isempty(duree), duree = zeros(4, 1); etat = false(4, 1); end
au_neutre = abs(imp(:) - imp_neutre) <= fenetre_armement_us;
duree = (duree + 1/f_trame_esc) .* au_neutre;
etat = etat | (duree >= t_armement) | (armement_actif == 0);
arme = double(etat);

== matlab function jumeau_banc_rw/Procédé/Jumeau Simscape/Capteurs de vitesse TCRT5000 x4/Mesure de la période ==
  data: theta input; w output; n_rayons parameter; T_tcrt parameter; t_arret_tcrt parameter
function w = mesure_periode(theta, n_rayons, T_tcrt, t_arret_tcrt)
% Carte TCRT5000 devant le disque : elle change d'état à chaque passage de rayon. L'ESP32 date chaque front et
% en tire la vitesse : un pas angulaire de 2 pi / n_rayons divisé par la durée entre deux fronts. Pas de signe.
% Le front est daté dans le pas de calcul par interpolation, comme le fait un chronomètre en microsecondes.
persistent k_prec th_prec t t_front w_mem
pas = 2*pi / n_rayons;
th = theta(:);
if isempty(k_prec)
    k_prec = floor(th / pas); th_prec = th; t = 0; t_front = -inf(4, 1); w_mem = zeros(4, 1);
end
k = floor(th / pas);
for j = 1:4
    if k(j) ~= k_prec(j)
        if k(j) > k_prec(j), th_f = k(j) * pas; else, th_f = k_prec(j) * pas; end   % dernier rayon franchi
        tf = t - T_tcrt + T_tcrt * (th_f - th_prec(j)) / (th(j) - th_prec(j));
        if isfinite(t_front(j)) && tf > t_front(j)
            w_mem(j) = abs(k(j) - k_prec(j)) * pas / (tf - t_front(j));
        end
        t_front(j) = tf;
    elseif t - t_front(j) > t_arret_tcrt
        w_mem(j) = 0;
    end
end
k_prec = k; th_prec = th; t = t + T_tcrt;
w = w_mem;

== matlab function jumeau_banc_rw/Procédé/Jumeau Webots/Trame de commande ==
  data: imp input; trame output; poussee input
function trame = trame_commande(imp, poussee)
% Trame de commande : celle de l'ESP32 du banc réel (A5 5A, 4 impulsions en µs en uint16, drapeaux, numéro), suivie, pour
% le jumeau seulement, de la poussée d'essai sur [roulis ; tangage] (2 nombres en simple précision, N.m), puis la somme.
persistent seq
if isempty(seq), seq = 0; end
t = zeros(21, 1, 'uint8');
t(1) = uint8(165); t(2) = uint8(90);
u = uint16(max(0, min(65535, round(imp(:)))));
t(3:10) = typecast(u, 'uint8');
t(11) = uint8(1);                              % bit 0 : marche
t(12) = uint8(seq);
t(13:20) = typecast(single(poussee(:)), 'uint8');
t(21) = uint8(mod(sum(double(t(1:20))), 256));
seq = mod(seq + 1, 256);
trame = t;

== matlab function jumeau_banc_rw/Procédé/Jumeau Webots/Envoi au procédé ==
  data: trame input
function envoi(trame)
% Envoie la trame de commande au procédé (liaison/pont_banc.m).
coder.extrinsic('pont_banc');
pont_banc('ecrire', trame);

== matlab function jumeau_banc_rw/Procédé/Jumeau Webots/Réception du procédé ==
  settings: updateMethod=DISCRETE  sampleTime=T_pont
  data: trame output
function trame = reception()
% Attend la trame de télémétrie du procédé (liaison/pont_banc.m) : Simulink et le jumeau restent au même instant.
coder.extrinsic('pont_banc');
trame = zeros(151, 1, 'uint8');
trame = pont_banc('lire');

== matlab function jumeau_banc_rw/Procédé/Jumeau Webots/Décodage de la télémétrie ==
  data: trame input uint8 size=[151 1]; euler output; gyro output; quat output; acc output; w_mes output; angles output; vitesses output; tr_min output; courants output; couples output; tensions output; rapports output; i_alim output; ok output
function [euler, gyro, quat, acc, w_mes, angles, vitesses, tr_min, courants, couples, tensions, rapports, i_alim, ok] = decodage(trame)
% Trame de télémétrie, la même que celle de l'ESP32 du banc réel : B5 5B, temps (ms), état, numéro,
% BNO055 en unités de ses registres (1/16 °, 1/16 °/s, 2^-14, 0,01 m/s²), 4 vitesses de roue (rad/s), somme.
% Le jumeau Webots ajoute ses grandeurs réelles (25 nombres en simple précision).
ok = double(trame(1) == 181 && trame(2) == 91 && mod(sum(double(trame(1:50))), 256) == double(trame(51)));
euler = double(typecast(trame(9:14), 'int16')) / 16;
gyro = double(typecast(trame(15:20), 'int16')) / 16;
quat = double(typecast(trame(21:28), 'int16')) / 2^14;
acc = double(typecast(trame(29:34), 'int16')) / 100;
w_mes = double(typecast(trame(35:50), 'single'));
v = double(typecast(trame(52:151), 'single'));
angles = v(1:2); vitesses = v(3:4); tr_min = v(5:8) * 60 / (2*pi);
courants = v(9:12); couples = v(13:16); tensions = v(17:20); rapports = v(21:24); i_alim = v(25);

== matlab function jumeau_banc_rw/Référence/Programme : polynômes de degré 5 ==
  data: t input; angle output; vitesse output; acceleration output; ref_t parameter; ref_roulis_deg parameter; ref_tangage_deg parameter; ref_duree parameter; q0_deg parameter
function [angle, vitesse, acceleration] = polynomes(t, ref_t, ref_roulis_deg, ref_tangage_deg, ref_duree, q0_deg)
% Référence programmée de roulis et de tangage. À chaque instant ref_t(i), le dispositif part vers le palier i
% [ref_roulis_deg(i) ; ref_tangage_deg(i)] et y arrive ref_duree plus tard, par un polynôme de degré 5 :
% vitesse et accélération nulles au départ et à l'arrivée. Avant ref_t(1) : la position de départ q0_deg.
% Sorties en degrés, degrés par seconde et degrés par seconde carrée, [roulis ; tangage].
cibles = [ref_roulis_deg(:) ref_tangage_deg(:)];
angle = q0_deg(:); vitesse = zeros(2, 1); acceleration = zeros(2, 1);
for i = 1:numel(ref_t)
    if t >= ref_t(i)
        if i == 1, a = q0_deg(:); else, a = cibles(i - 1, :).'; end
        b = cibles(i, :).';
        s = min((t - ref_t(i)) / ref_duree, 1);
        angle = a + (b - a) * (10*s^3 - 15*s^4 + 6*s^5);
        vitesse = (b - a) * (30*s^2 - 60*s^3 + 30*s^4) / ref_duree;
        acceleration = (b - a) * (60*s - 180*s^2 + 120*s^3) / ref_duree^2;
    end
end
